simulink model "lab8_model"  (R2025b)
settings: Solver=VariableStepAuto  StartTime=0.0  StopTime=10.0  RelTol=1e-3
model workspace (MAT data in the model file):
  Kd_sim = Simulink.Parameter
  Kd_sim.Value = 0
  Kd_sim.Complexity = 'real'
  Kd_sim.Dimensions = [1 1]
  Kd_sim.DataType = 'auto'
  Ki_sim = Simulink.Parameter
  Ki_sim.Value = 0
  Ki_sim.Complexity = 'real'
  Ki_sim.Dimensions = [1 1]
  Ki_sim.DataType = 'auto'
  Kp_sim = Simulink.Parameter
  Kp_sim.Value = 0
  Kp_sim.Complexity = 'real'
  Kp_sim.Dimensions = [1 1]
  Kp_sim.DataType = 'auto'
  sys = Simulink.Parameter
  sys.Complexity = 'real'
  sys.Dimensions = [0 0]
  sys.DataType = 'auto'
undefined symbols (not defined in the file or in its folder): ref
libraries: cstblocks x1
settings Model: Creator=grantdahl  LastModifiedBy=grantdahl

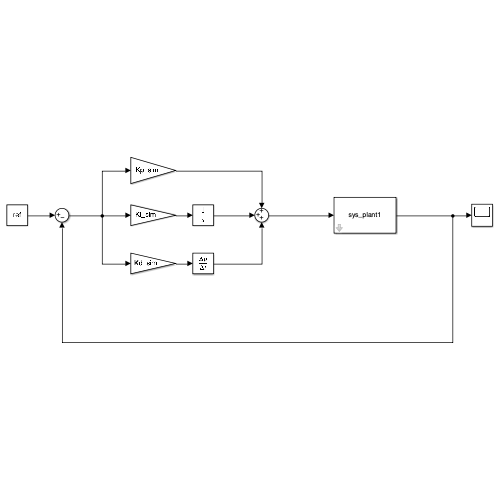
[thumbnail: Simulink's stored preview of the top-level diagram]
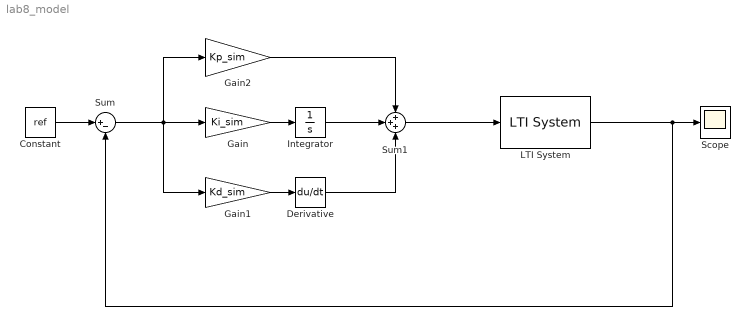
== system lab8_model ==
  Constant : Constant  Value=ref
  Derivative : Derivative
  Gain : Gain  Gain=Ki_sim
  Gain1 : Gain  Gain=Kd_sim
  Gain2 : Gain  Gain=Kp_sim
  Integrator : Integrator
  LTI System : cstblocks/LTI System  sys=sys_plant1  IC=[]  PadeOrder=0
  Scope : Scope
      settings: ActiveDisplayYMinimum=-71.589988796085876  ActiveDisplayYMaximum=644.309899164773
  Sum : Sum  Inputs=|+-
  Sum1 : Sum  Inputs=+++
  wires:
  Sum1/1 -> LTI System/1
  LTI System/1 -> Scope/1, Sum/2
  Constant/1 -> Sum/1
  Gain1/1 -> Derivative/1
  Gain2/1 -> Sum1/1
  Sum/1 -> Gain2/1, Gain1/1, Gain/1
  Derivative/1 -> Sum1/3
  Gain/1 -> Integrator/1
  Integrator/1 -> Sum1/2
